simulink model "PDW_Controller"  (R2022b)
settings: Solver=FixedStepDiscrete  StartTime=0.0  StopTime=10.0  FixedStep=0.02  RelTol=1e-3
libraries: simulink x10
settings Model: Creator=chaym  LastModifiedBy=chaym
settings OptimizationCC: DefaultParameterBehavior=Inlined  EnhancedBackFolding=on  PassReuseOutputArgsAs=Individual arguments  ZeroExternalMemoryAtStartup=off  ZeroInternalMemoryAtStartup=off  OptimizeBlockOrder=speed  DifferentSizesBufferReuse=on  OptimizationCustomize=off  EfficientTunableParamExpr=on
settings DebuggingCC: ParameterPrecisionLossMsg=none  ParameterTunabilityLossMsg=error
settings SFSimCC: MATLABDynamicMemAlloc=off
settings RTWCC: Description=AUTOSAR  SystemTargetFile=autosar.tlc  GenCodeOnly=on  TemplateMakefile=ert_default_tmf
settings CodeAppCC: ForceParamTrailComments=on  IgnoreCustomStorageClasses=off  OperatorAnnotations=on  SimulinkDataObjDesc=on  SFDataObjDesc=on  InsertBlockDesc=on
settings STFCustomTargetCC: TargetLangStandard=C99 (ISO)  MultiwordLength=256  ParMdlRefBuildCompliant=on  CompOptLevelCompliant=on  IncludeMdlTerminateFcn=off  CombineOutputUpdateFcns=on  SuppressErrorStatus=on  ERTCustomFileBanners=on  SupportNonFinite=off  SupportComplex=off  SupportContinuousTime=off  SupportNonInlinedSFcns=off  RemoveResetFunc=on  MATLABClassNameForMDSCustomization=Simulink.SoftwareTarget.ERTCustomization  AutosarCompliant=on  UseToolchainInfoCompliant=on  LookupTableObjectStructAxisOrder=2,1,3,4,...  LUTObjectStructOrderEvenSpacing=Size,Table,Breakpoints  SystemTargetFile=autosar.tlc
settings ERTTargetCC: TargetLangStandard=C99 (ISO)  ConcurrentExecutionCompliant=off  IncludeMdlTerminateFcn=off  SuppressErrorStatus=on  SupportNonFinite=off  SupportComplex=off  ModelStepFunctionPrototypeControlCompliant=off  CPPClassGenCompliant=off  AutosarCompliant=on  LookupTableObjectStructAxisOrder=2,1,3,4,...  LUTObjectStructOrderEvenSpacing=Size,Table,Breakpoints  InlinedParameterPlacement=NonHierarchical  ERTCustomFileTemplate=example_file_process.tlc

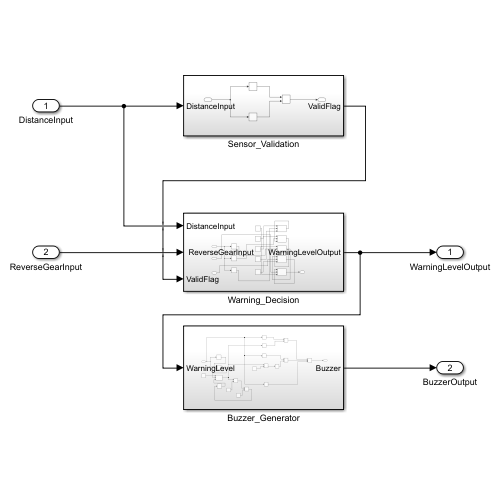
[thumbnail: Simulink's stored preview of the top-level diagram]
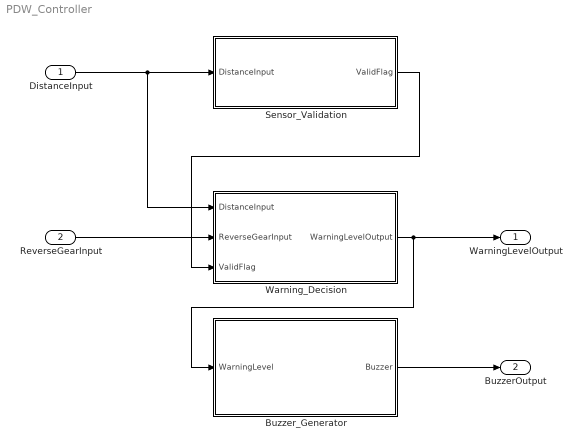
== system PDW_Controller ==
  DistanceInput : Inport  OutDataTypeStr=single  PortDimensions=1  SampleTime=0.02
  ReverseGearInput : Inport  Port=2  OutDataTypeStr=boolean  PortDimensions=1  SampleTime=0.02
  Buzzer_Generator : Subsystem
  Sensor_Validation : Subsystem
  Warning_Decision : Subsystem
  WarningLevelOutput : Outport
  BuzzerOutput : Outport  Port=2
  wires:
  DistanceInput/1 -> Sensor_Validation/1(DistanceInput), Warning_Decision/1(DistanceInput)
  ReverseGearInput/1 -> Warning_Decision/2("\tReverseGearInput")
  Sensor_Validation/1(ValidFlag) -> Warning_Decision/3(ValidFlag)
  Warning_Decision/1(WarningLevelOutput) -> Buzzer_Generator/1(WarningLevel), WarningLevelOutput/1
  Buzzer_Generator/1(Buzzer) -> BuzzerOutput/1

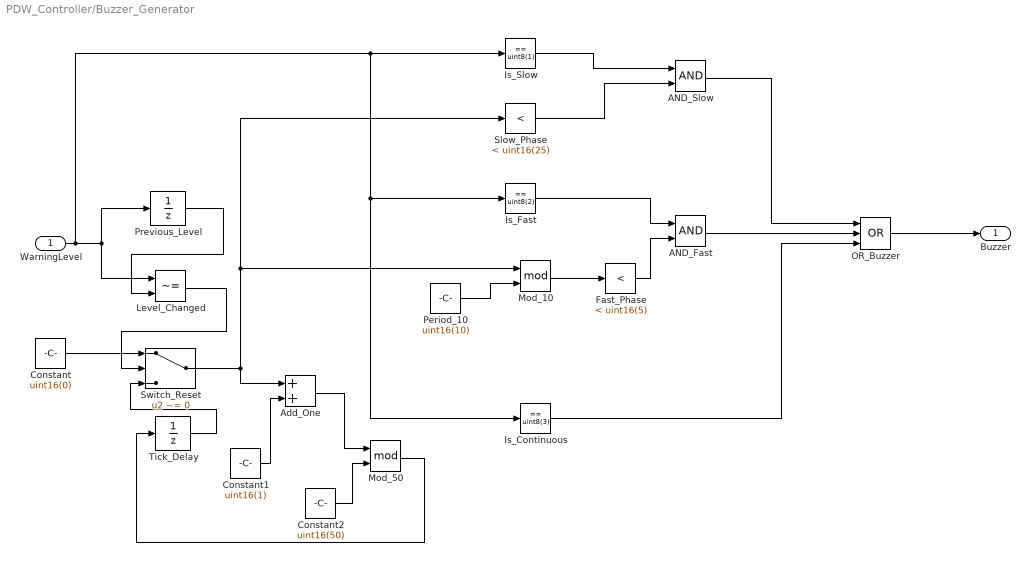
== system PDW_Controller/Buzzer_Generator ==
  WarningLevel : Inport
  AND_Fast : Logic  AllPortsSameDT=off  OutDataTypeStr=boolean
  AND_Slow : Logic  AllPortsSameDT=off  OutDataTypeStr=boolean
  Add_One : Sum
  Constant : Constant  Value=uint16(0)  OutDataTypeStr=uint16
  Constant1 : Constant  Value=uint16(1)
  Constant2 : Constant  Value=uint16(50)
  Fast_Phase : simulink/Logic and Bit Operations/Compare To Constant  relop=<  const=uint16(5)  OutDataTypeStr=boolean
  Is_Continuous : simulink/Logic and Bit Operations/Compare To Constant  relop===  const=uint8(3)  OutDataTypeStr=boolean
  Is_Fast : simulink/Logic and Bit Operations/Compare To Constant  relop===  const=uint8(2)  OutDataTypeStr=boolean
  Is_Slow : simulink/Logic and Bit Operations/Compare To Constant  relop===  const=uint8(1)  OutDataTypeStr=boolean
  Level_Changed : RelationalOperator  Operator=~=  OutDataTypeStr=boolean  RndMeth=Simplest  InputSameDT=off
  Mod_10 : Math  Operator=mod
  Mod_50 : Math  Operator=mod
  OR_Buzzer : Logic  Operator=OR  Inputs=3  AllPortsSameDT=off  OutDataTypeStr=boolean
  Period_10 : Constant  Value=uint16(10)
  Previous_Level : UnitDelay  InitialCondition=uint8(0)  SampleTime=0.02  HasFrameUpgradeWarning=on
  Slow_Phase : simulink/Logic and Bit Operations/Compare To Constant  relop=<  const=uint16(25)  OutDataTypeStr=boolean
  Switch_Reset : Switch  Criteria=u2 ~= 0  SaturateOnIntegerOverflow=off  InputSameDT=off
  Tick_Delay : UnitDelay  InitialCondition=uint16(0)  SampleTime=0.02  HasFrameUpgradeWarning=on
  Buzzer : Outport  OutDataTypeStr=boolean
  wires:
  WarningLevel/1 -> Is_Continuous/1, Is_Fast/1, Is_Slow/1, Previous_Level/1, Level_Changed/1
  Previous_Level/1 -> Level_Changed/2
  Constant/1 -> Switch_Reset/1
  Level_Changed/1 -> Switch_Reset/2
  Switch_Reset/1 -> Slow_Phase/1, Mod_10/1, Add_One/1
  Tick_Delay/1 -> Switch_Reset/3
  Constant1/1 -> Add_One/2
  Add_One/1 -> Mod_50/1
  Constant2/1 -> Mod_50/2
  Mod_50/1 -> Tick_Delay/1
  Is_Slow/1 -> AND_Slow/1
  Slow_Phase/1 -> AND_Slow/2
  Mod_10/1 -> Fast_Phase/1
  Fast_Phase/1 -> AND_Fast/2
  Is_Fast/1 -> AND_Fast/1
  OR_Buzzer/1 -> Buzzer/1
  AND_Slow/1 -> OR_Buzzer/1
  AND_Fast/1 -> OR_Buzzer/2
  Is_Continuous/1 -> OR_Buzzer/3
  Period_10/1 -> Mod_10/2

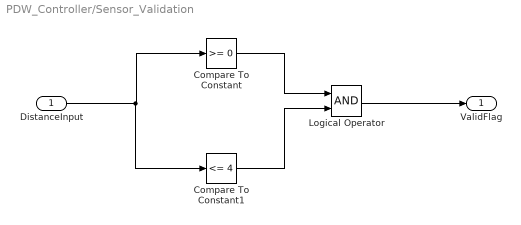
== system PDW_Controller/Sensor_Validation ==
  DistanceInput : Inport
  Compare To Constant : simulink/Logic and Bit Operations/Compare To Constant  relop=>=  const=0  OutDataTypeStr=boolean
  Compare To Constant1 : simulink/Logic and Bit Operations/Compare To Constant  relop=<=  const=4  OutDataTypeStr=boolean
  Logical Operator : Logic  AllPortsSameDT=off  OutDataTypeStr=boolean
  ValidFlag : Outport
  wires:
  Logical Operator/1 -> ValidFlag/1
  DistanceInput/1 -> Compare To Constant1/1, Compare To Constant/1
  Compare To Constant/1 -> Logical Operator/1
  Compare To Constant1/1 -> Logical Operator/2

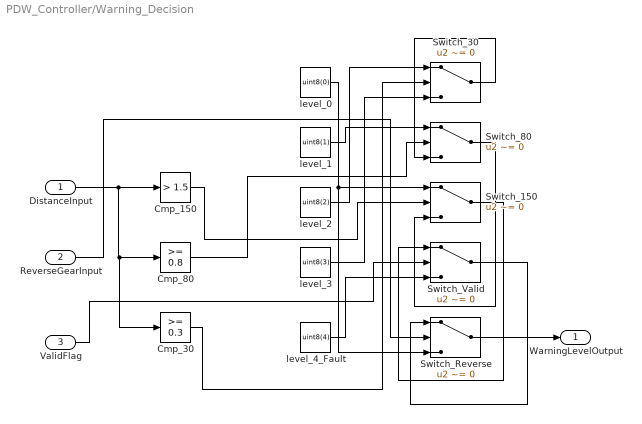
== system PDW_Controller/Warning_Decision ==
  DistanceInput : Inport
  "\tReverseGearInput" : Inport  Port=2
  ValidFlag : Inport  Port=3
  Cmp_150 : simulink/Logic and Bit Operations/Compare To Constant  relop=>  const=1.5  OutDataTypeStr=boolean
  Cmp_30 : simulink/Logic and Bit Operations/Compare To Constant  relop=>=  const=0.3  OutDataTypeStr=boolean
  Cmp_80 : simulink/Logic and Bit Operations/Compare To Constant  relop=>=  const=0.8  OutDataTypeStr=boolean
  Switch_150 : Switch  Criteria=u2 ~= 0  SaturateOnIntegerOverflow=off  InputSameDT=off
  Switch_30 : Switch  Criteria=u2 ~= 0  SaturateOnIntegerOverflow=off  InputSameDT=off
  Switch_80 : Switch  Criteria=u2 ~= 0  SaturateOnIntegerOverflow=off  InputSameDT=off
  Switch_Reverse : Switch  Criteria=u2 ~= 0  SaturateOnIntegerOverflow=off  InputSameDT=off
  Switch_Valid : Switch  Criteria=u2 ~= 0  SaturateOnIntegerOverflow=off  InputSameDT=off
  level_0 : Constant  Value=uint8(0)
  level_1 : Constant  Value=uint8(1)
  level_2 : Constant  Value=uint8(2)
  level_3 : Constant  Value=uint8(3)
  level_4_Fault : Constant  Value=uint8(4)
  WarningLevelOutput : Outport
  wires:
  DistanceInput/1 -> Cmp_30/1, Cmp_80/1, Cmp_150/1
  Cmp_30/1 -> Switch_30/2
  level_2/1 -> Switch_30/1
  level_3/1 -> Switch_30/3
  Cmp_80/1 -> Switch_80/2
  level_1/1 -> Switch_80/1
  Switch_30/1 -> Switch_80/3
  Cmp_150/1 -> Switch_150/2
  level_0/1 -> Switch_Reverse/3, Switch_150/1
  Switch_80/1 -> Switch_150/3
  ValidFlag/1 -> Switch_Valid/2
  Switch_150/1 -> Switch_Valid/1
  level_4_Fault/1 -> Switch_Valid/3
  "\tReverseGearInput"/1 -> Switch_Reverse/2
  Switch_Valid/1 -> Switch_Reverse/1
  Switch_Reverse/1 -> WarningLevelOutput/1
